simulink model "FDM"  (R2026a)
settings: Solver=FixedStepDiscrete  StopTime=Tsim  FixedStep=Ts
InitFcn:
  | tx_params
values from neighbouring files (symbols this model uses):
  K_FDM = 1/3    (= 0.333333333333)    [tx_params.m]
  Ts = 1/Fs    (= 2e-07)    [tx_params.m]
libraries: commanapbnd3 x3
settings Model: Creator=fel.sanchez  LastModifiedBy=User

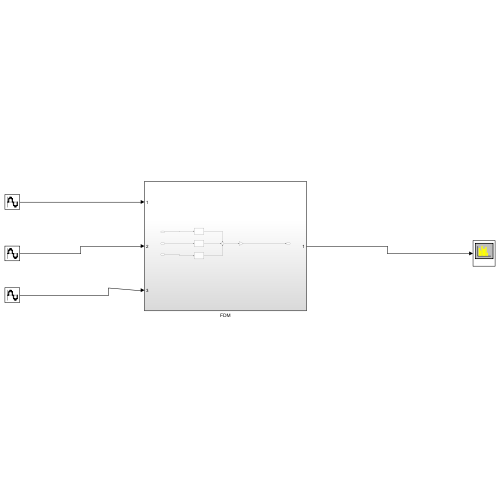
[thumbnail: Simulink's stored preview of the top-level diagram]
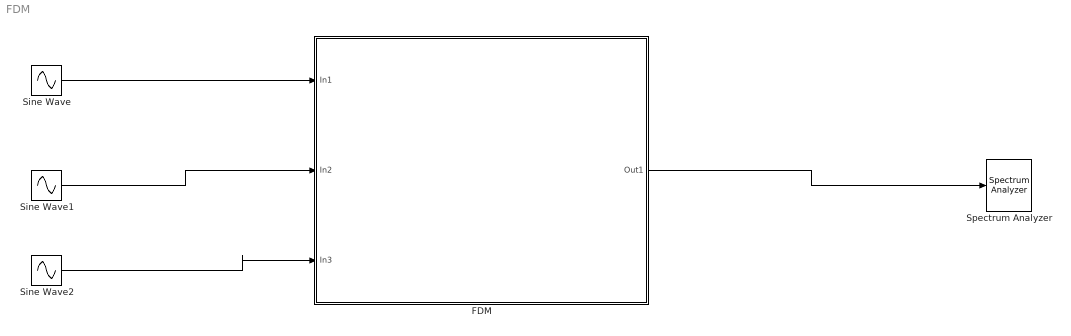
== system FDM ==
  FDM : Subsystem
  Sine Wave : Sin  Frequency=2*pi*1000  SampleTime=Ts
  Sine Wave1 : Sin  Frequency=2*pi*3000  SampleTime=Ts
  Sine Wave2 : Sin  Frequency=2*pi*6000  SampleTime=Ts
  Spectrum Analyzer : SpectrumAnalyzer  Method=Welch  PlotAsTwoSidedSpectrum=off  AveragingMethod=Exponential
  wires:
  Sine Wave/1 -> FDM/1(In1)
  Sine Wave1/1 -> FDM/2(In2)
  Sine Wave2/1 -> FDM/3(In3)
  FDM/1(Out1) -> Spectrum Analyzer/1

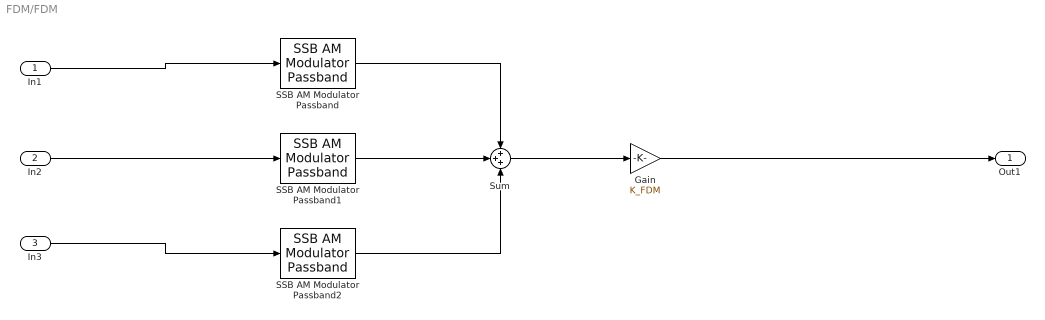
== system FDM/FDM ==
  In1 : Inport
  In2 : Inport  Port=2
  In3 : Inport  Port=3
  Gain : Gain  Gain=K_FDM
  SSB AM Modulator Passband : commanapbnd3/SSB AM Modulator Passband  Fc=fc1  Ph=0  Sd=Upper  Ho=Nh
  SSB AM Modulator Passband1 : commanapbnd3/SSB AM Modulator Passband  Fc=fc2  Ph=0  Sd=Upper  Ho=Nh
  SSB AM Modulator Passband2 : commanapbnd3/SSB AM Modulator Passband  Fc=fc3  Ph=0  Sd=Upper  Ho=Nh
  Sum : Sum  Inputs=+++
  Out1 : Outport
  wires:
  SSB AM Modulator Passband1/1 -> Sum/2
  SSB AM Modulator Passband2/1 -> Sum/3
  Sum/1 -> Gain/1
  SSB AM Modulator Passband/1 -> Sum/1
  Gain/1 -> Out1/1
  In3/1 -> SSB AM Modulator Passband2/1
  In2/1 -> SSB AM Modulator Passband1/1
  In1/1 -> SSB AM Modulator Passband/1
